simulink model "ac1_2025a"  (R2025a)
settings: Solver=VariableStepAuto  StartTime=0.0  StopTime=3  RelTol=1e-3
model workspace (MAT data in the model file):
  p = 0.0002
libraries: spsVoltageMeasurementLib x7, spsACVoltageSourceLib x3, eeGeneralControl x3, eePwmGeneratorTwoLevel x2, spsThreePhaseSineGeneratorLib x2, spsUniversalBridgeLib x2, spsAsynchronousMachineSIUnitsLib x1, spsGroundLib x1, eePowerMeasurement x1, simulink x1, spsSeriesRLCBranchLib x1, spsThreePhaseVIMeasurementLib x1
settings Model: Creator=adith  LastModifiedBy=DELL

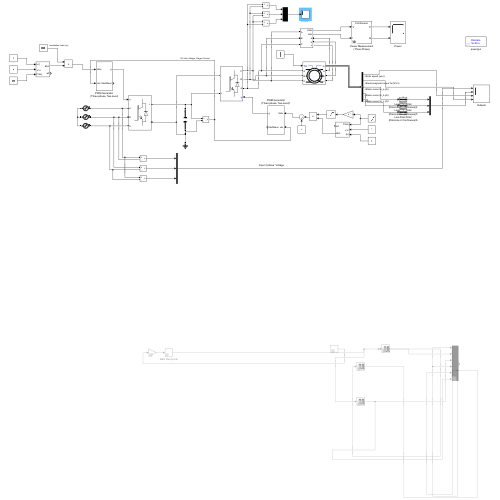
[thumbnail: Simulink's stored preview of the top-level diagram]
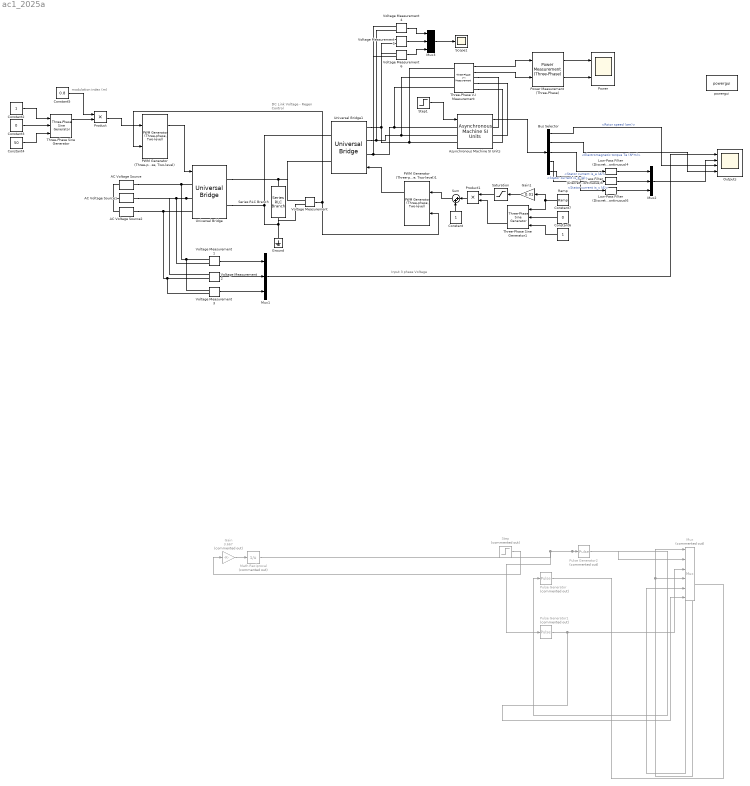
== system ac1_2025a ==
  note: Input 3 phase Voltage
  note: modulation index (m)
  note: DC Link Voltage - Regen Control
  AC Voltage Source : spsACVoltageSourceLib/AC Voltage Source  Amplitude=400  Phase=0  Frequency=50  SampleTime=0  Measurements=None  BusType=swing  Pref=10e3  Qref=0  Qmin=-inf  Qmax=+inf
  AC Voltage Source1 : spsACVoltageSourceLib/AC Voltage Source  Amplitude=400  Phase=120  Frequency=50  SampleTime=0  Measurements=None  BusType=swing  Pref=10e3  Qref=0  Qmin=-inf  Qmax=+inf
  AC Voltage Source2 : spsACVoltageSourceLib/AC Voltage Source  Amplitude=400  Phase=-120  Frequency=50  SampleTime=0  Measurements=None  BusType=swing  Pref=10e3  Qref=0  Qmin=-inf  Qmax=+inf
  Asynchronous Machine SI Units : spsAsynchronousMachineSIUnitsLib/Asynchronous Machine SI Units  RotorType=Wound  PresetModel=No  MechanicalLoad=Torque Tm  ShowDetailedParameters=on  ReferenceFrame=Rotor  Units=SI  MeasurementBus=off  NominalParameters=[1.845e+04 400 50]  VoltageRatio=1  Stator=[0.5968 0.0003495]  Rotor=[0.6258 0.005473]  Cage1=[0.4155 0.002066]  Cage2=[0.4168 0.0003495]  Lm=0.0354  Mechanical=[0.05 0.005879 2]  PolePairs=2  InitialConditions=[0 0 0 0 0 0 0 0]  SimulateSaturation=off  Saturation=[14.03593122, 27.81365428, 53.79336849, 72.68890987, 97.98006896, 148.6815601, 215.7428561, 302.9841135, 428.7778367 ; 230, 322, 414, 460, 506, 552, 598, 644, 690]  LoadFlowParameters=1492000  TsPowergui=0  TsBlock=-1  IterativeModel=Trapezoidal non iterative  IterativeDiscreteModel=Trapezoidal non iterative  Pmec=1.492e+006
  Bus Selector : BusSelector  OutputSignals=Mechanical.Rotor speed (wm),Mechanical.Electromagnetic torque Te (N*m),Stator measurements.Stator current is_a (A),Stator measurements.Stator current is_b (A),Stator measurements.Stator current is_c (A)
  Constant : Constant
  Constant2 : Constant
  Constant3 : Constant  Value=0
  Constant4 : Constant  Value=50
  Constant5 : Constant  Value=0.8
  Constant6 : Constant
  Constant7 : Constant  Value=0
  Gain : Gain  Commented=on  Gain=3.667
  Gain1 : Gain  Gain=0.01
  Ground : spsGroundLib/Ground  LConnTagsString=a
  Low-Pass Filter (Discrete or Continuous)4 : eeGeneralControl/Low-Pass Filter (Discrete or Continuous)  K=1  T=0.001  B=inf  A=-inf  init_option=Inherited from block input  x0=0  Ts=-1
  Low-Pass Filter (Discrete or Continuous)5 : eeGeneralControl/Low-Pass Filter (Discrete or Continuous)  K=1  T=0.001  B=inf  A=-inf  init_option=Inherited from block input  x0=0  Ts=-1
  Low-Pass Filter (Discrete or Continuous)6 : eeGeneralControl/Low-Pass Filter (Discrete or Continuous)  K=1  T=0.001  B=inf  A=-inf  init_option=Inherited from block input  x0=0  Ts=-1
  Math Reciprocal : Math  Commented=on  Operator=reciprocal  SignedPower=on
  Mux : Mux  Commented=on  Inputs=6
  Mux1 : Mux  Inputs=3
  Mux2 : Mux  Inputs=3
  Mux3 : Mux  Inputs=3
  Outputs : Scope  NumInputPorts=4
      settings: ActiveDisplayYMinimum=-866.0254037844611  ActiveDisplayYMaximum=866.0254037844611
  "PWM Generator (Three-phase, Two-level)" : eePwmGeneratorTwoLevel/PWM Generator (Three-phase, Two-level)  PWMMode=Continuous PWM (CPWM)  CPWMMode=SPWM: sinusoidal PWM  DPWMMode=60 DPWM: 60 degree discontinuous PWM  fsw=1e3  Ts=5e-6
      settings: LibrarySourceBlock=|
      | ee_sl_lib/Pulse Width
      | Modulation/PWM Generator
      | (Three-phase, Two-level)
  "PWM Generator (Three-phase, Two-level)1" : eePwmGeneratorTwoLevel/PWM Generator (Three-phase, Two-level)  PWMMode=Continuous PWM (CPWM)  CPWMMode=SPWM: sinusoidal PWM  DPWMMode=60 DPWM: 60 degree discontinuous PWM  fsw=1e3  Ts=5e-6
      settings: LibrarySourceBlock=|
      | ee_sl_lib/Pulse Width
      | Modulation/PWM Generator
      | (Three-phase, Two-level)
  Power : Scope  NumInputPorts=2
      settings: ActiveDisplayYMinimum=-0.056520972602042086  ActiveDisplayYMaximum=0.11555867027126868
  Power Measurement (Three-Phase) : eePowerMeasurement/Power Measurement (Three-Phase)  LabelModeActiveChoice=Continuous  F=60  K=[0 1 2 3]  Seq=Positive  Ts=0
  Product : Product
  Product1 : Product
  Pulse Generator : DiscretePulseGenerator  Commented=on  PulseType=Time based  TimeSource=Use external signal  Period=0.0002  PulseWidth=50
  Pulse Generator1 : DiscretePulseGenerator  Commented=on  PulseType=Time based  TimeSource=Use external signal  Period=0.0002  PulseWidth=50  PhaseDelay=0.01111
  Pulse Generator2 : DiscretePulseGenerator  Commented=on  PulseType=Time based  TimeSource=Use external signal  Period=0.0002  PulseWidth=50  PhaseDelay=0.00556
  Ramp : simulink/Sources/Ramp  slope=40  start=0  InitialOutput=0
  Saturation : Saturate  UpperLimit=1  LowerLimit=0
  Scope1 : Scope
      settings: ActiveDisplayYMinimum=-56.432970405149717  ActiveDisplayYMaximum=443.13970829924671  DataLoggingVariableName=ScopeData3
  Series RLC Branch : spsSeriesRLCBranchLib/Series RLC Branch  LConnTagsString=__new0  RConnTagsString=__new0  BranchType=C  Resistance=1  Inductance=1e-3  SetiL0=off  InitialCurrent=0  Capacitance=1e-6  Setx0=off  InitialVoltage=0  Measurements=None
  Step : Step  Commented=on  Time=5  Before=60  After=20  SampleTime=0
  Step1 : Step  Time=0.5  After=2  SampleTime=0
  Sum : Sum  Inputs=|++
  Three-Phase Sine Generator : spsThreePhaseSineGeneratorLib/Three-Phase Sine Generator  Ts=0
      settings: LibrarySourceBlock=|
      | sps_lib/Sources/Signal Generator Sources/Three-Phase
      | Sine Generator
  Three-Phase Sine Generator1 : spsThreePhaseSineGeneratorLib/Three-Phase Sine Generator  Ts=0
      settings: LibrarySourceBlock=|
      | sps_lib/Sources/Signal Generator Sources/Three-Phase
      | Sine Generator
  Three-Phase V-I Measurement : spsThreePhaseVIMeasurementLib/Three-Phase V-I Measurement  VoltageMeasurement=phase-to-ground  SetLabelV=off  LabelV=Vabc  Vpu=off  VpuLL=off  CurrentMeasurement=yes  SetLabelI=off  LabelI=Iabc  Ipu=off  Pbase=100e6  Vbase=500e3  OutputType=Complex  PhasorSimulation=off  PSBequivalent=0
  Universal Bridge : spsUniversalBridgeLib/Universal Bridge  Arms=3  SnubberResistance=1e5  SnubberCapacitance=inf  Device=IGBT / Diodes  Ron=1e-3  Lon=0  ForwardVoltages="[  0  0  ]"  ForwardVoltage=0  GTOparameters=[ 10e-6 , 20e-6 ]  IGBTparameters=[ 1e-6 , 2e-6 ]  Measurements=None  Measurements_2=None  converterType=Rectifier
  Universal Bridge1 : spsUniversalBridgeLib/Universal Bridge  Arms=3  SnubberResistance=1e5  SnubberCapacitance=inf  Device=IGBT / Diodes  Ron=1e-3  Lon=0  ForwardVoltages="[  0  0  ]"  ForwardVoltage=0  GTOparameters=[ 10e-6 , 20e-6 ]  IGBTparameters=[ 1e-6 , 2e-6 ]  Measurements=None  Measurements_2=None  converterType=Rectifier
  Voltage Measurement{,1..6} (7 alike) : spsVoltageMeasurementLib/Voltage Measurement  PhasorSimulation=off  OutputType=Complex  PSBequivalent=0
  powergui : sps_lib/powergui  Priority=1  SimulationMode=Discrete  SampleTime=5e-6  frequency=60  Iterations=50  frequencyindice=50  Pbase=100e6  ErrMax=1e-4  UnitsV=kV  UnitsW=MW  buscounter=0  FunctionMessages=off  echomessages=off  EnableUseOfTLC=off  CurrentSourceSwitches=off  DisableSnubberDevices=off  DisableRonSwitches=off  DisableVfSwitches=off  DisplayEquations=off  AutomaticDiscreteSolvers=off  SolverType=Tustin/Backward Euler (TBE)  Interpol=off  ExternalGateDelay=off  methode=off  Ts=100  x0status=blocks  SPID=on  SwTol=0  HookPort=off  NonlinearTolerance=1e-4  nMaxIteration=100  ContinueOnMaxIteration=off  RestoreLinks=warning  ResistiveCurrentMeasurement=off  Frange=[0:2:500]  Ylog=off  Xlog=on  ShowGrid=off  save=off  variable=ZData  structure=0  ZoomFFT=off  StartTime=0.0  cycles=1  DisplayStyle=1  fundamental=60  FreqAxis=off  MaxFrequency=1000  frequencyindicesteady=1  RmsSteady=1  display=off
  wires:
  Step1/1 -> Asynchronous Machine SI Units/1
  Step/1 -> Gain/1
  Asynchronous Machine SI Units/1 -> Bus Selector/1
  Bus Selector/1 -> Outputs/3  "<Rotor speed (wm)>"
  Pulse Generator/1 -> Mux/5, Mux/1, Mux/4
  Pulse Generator2/1 -> Mux/2
  Pulse Generator1/1 -> Mux/6, Mux/3
  Gain/1 -> Math Reciprocal/1
  Math Reciprocal/1 -> Pulse Generator/1, Pulse Generator2/1, Pulse Generator1/1
  Three-Phase Sine Generator/1 -> Product/2
  "PWM Generator (Three-phase, Two-level)"/1 -> Universal Bridge/1
  Voltage Measurement/1 -> "PWM Generator (Three-phase, Two-level)1"/2, "PWM Generator (Three-phase, Two-level)"/2
  Product/1 -> "PWM Generator (Three-phase, Two-level)"/1
  Constant2/1 -> Three-Phase Sine Generator/1
  Constant3/1 -> Three-Phase Sine Generator/2
  Constant4/1 -> Three-Phase Sine Generator/3
  Ramp/1 -> Three-Phase Sine Generator1/3, Gain1/1
  Constant7/1 -> Three-Phase Sine Generator1/2
  Constant6/1 -> Three-Phase Sine Generator1/1
  "PWM Generator (Three-phase, Two-level)1"/1 -> Universal Bridge1/1
  Gain1/1 -> Saturation/1
  Three-Phase Sine Generator1/1 -> Product1/2
  Saturation/1 -> Product1/1
  Product1/1 -> Sum/1
  Constant/1 -> Sum/2
  Sum/1 -> "PWM Generator (Three-phase, Two-level)1"/1
  Bus Selector/2 -> Outputs/4  "<Electromagnetic torque Te (N*m)>"
  Three-Phase V-I Measurement/1 -> Power Measurement (Three-Phase)/1
  Power Measurement (Three-Phase)/2 -> Power/2
  Power Measurement (Three-Phase)/1 -> Power/1
  Three-Phase V-I Measurement/2 -> Power Measurement (Three-Phase)/2
  Bus Selector/5 -> Low-Pass Filter (Discrete or Continuous)6/1  "<Stator current is_c (A)>"
  Mux2/1 -> Outputs/2
  Low-Pass Filter (Discrete or Continuous)4/1 -> Mux2/1
  Low-Pass Filter (Discrete or Continuous)5/1 -> Mux2/2
  Low-Pass Filter (Discrete or Continuous)6/1 -> Mux2/3
  Bus Selector/3 -> Low-Pass Filter (Discrete or Continuous)4/1  "<Stator current is_a (A)>"
  Bus Selector/4 -> Low-Pass Filter (Discrete or Continuous)5/1  "<Stator current is_b (A)>"
  Voltage Measurement1/1 -> Mux1/1
  Voltage Measurement2/1 -> Mux1/2
  Voltage Measurement3/1 -> Mux1/3
  Mux1/1 -> Outputs/1
  Constant5/1 -> Product/1
  Mux3/1 -> Scope1/1
  Voltage Measurement4/1 -> Mux3/1
  Voltage Measurement5/1 -> Mux3/2
  Voltage Measurement6/1 -> Mux3/3
  connections:
  Voltage Measurement1/LConn1 -- Voltage Measurement3/LConn1 -- AC Voltage Source/RConn1 -- Universal Bridge/LConn1
  Universal Bridge/LConn2 -- AC Voltage Source1/RConn1 -- Voltage Measurement2/LConn1 -- Voltage Measurement1/LConn2
  Voltage Measurement2/LConn2 -- Voltage Measurement3/LConn2 -- AC Voltage Source2/RConn1 -- Universal Bridge/LConn3
  Universal Bridge/RConn1 -- Universal Bridge1/RConn1 -- Voltage Measurement/LConn1 -- Series RLC Branch/LConn1
  Universal Bridge1/LConn3 -- Voltage Measurement5/LConn2 -- Voltage Measurement6/LConn1 -- Three-Phase V-I Measurement/LConn1 -- Asynchronous Machine SI Units/LConn3
  Universal Bridge1/LConn2 -- Voltage Measurement4/LConn2 -- Voltage Measurement5/LConn1 -- Three-Phase V-I Measurement/LConn2 -- Asynchronous Machine SI Units/LConn2
  Universal Bridge1/LConn1 -- Voltage Measurement6/LConn2 -- Voltage Measurement4/LConn1 -- Three-Phase V-I Measurement/LConn3 -- Asynchronous Machine SI Units/LConn1
  Universal Bridge/RConn2 -- Universal Bridge1/RConn2 -- Voltage Measurement/LConn2 -- Series RLC Branch/RConn1 -- Ground/LConn1
  Three-Phase V-I Measurement/RConn1 -- Asynchronous Machine SI Units/RConn1
  Three-Phase V-I Measurement/RConn2 -- Asynchronous Machine SI Units/RConn2
  Three-Phase V-I Measurement/RConn3 -- Asynchronous Machine SI Units/RConn3
  AC Voltage Source2/LConn1 -- AC Voltage Source/LConn1 -- AC Voltage Source1/LConn1
